simulink model "pendolo_simulink"  (R2026a)
settings: Solver=ode45  StopTime=30  MaxStep=0.01
values from neighbouring files (symbols this model uses):
  b = 0.2    [parametri_pendolo.m]
  ell = L/2    (= 0.5)    [parametri_pendolo.m]
  g = 9.81    [parametri_pendolo.m]
  I = m*L^2/3    (= 0.333333333333)    [parametri_pendolo.m]
  m = 1    [parametri_pendolo.m]
  omega0 = 0    [parametri_pendolo.m]
  theta0 = pi - 0.01    (= 3.13159265359)    [parametri_pendolo.m]
settings Model: Creator=bellu  LastModifiedBy=bellu

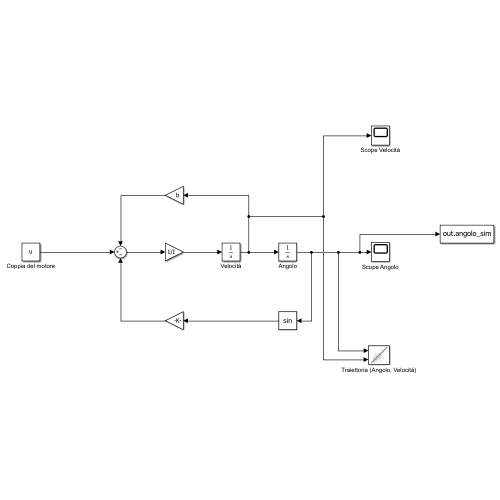
[thumbnail: Simulink's stored preview of the top-level diagram]
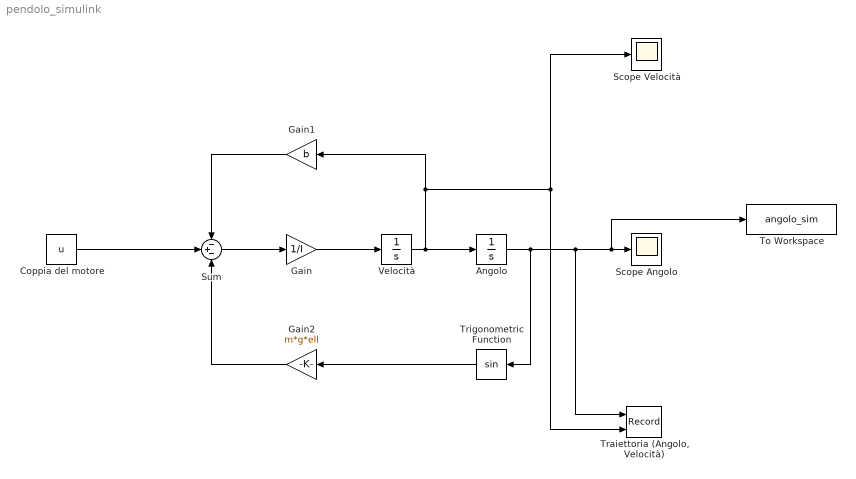
== system pendolo_simulink ==
  Angolo : Integrator  InitialCondition=theta0
  Coppia del motore : Constant  Value=u
  Gain : Gain  Gain=1/I
  Gain1 : Gain  Gain=b
  Gain2 : Gain  Gain=m*g*ell
  Scope Angolo : Scope
      settings: ActiveDisplayYMinimum=-3.4958404131067238  ActiveDisplayYMaximum=5.4026268178633838
  Scope Velocità : Scope
      settings: ActiveDisplayYMinimum=-7.8449946519179914  ActiveDisplayYMaximum=6.1158449546451417
  Sum : Sum  Inputs=-+-
  To Workspace : ToWorkspace  VariableName=angolo_sim  SaveFormat=Timeseries  SampleTime=-1
  "Traiettoria (Angolo, Velocità)" : Record  NumPorts=2.0  FileSettingsInternal="{\"entries\":[{\"content\":{\"excelSettings\":{\"content\":{},\"type\":\"Streamout.ExcelSettings\"},\"parquetSettings\":{\"content\":{},\"type\":\"Streamout.ParquetSettings\"}},\"type\":\"Streamout.FileSettingStorage\",\"uuid\":\"\"}],\"packageUris\":[\"http:\\/\\/schema.mathworks.com\\/mf0\\/streamout_blocks\\/R2020a\"],\"version\":\"1.0\"}"  FrameSettings=[0, 0]  Layout=[1 1]  SignalsInternal="{\"entries\":[{\"content\":{\"signals\":[{\"content\":{\"blockPath\":[],\"dimensions\":[1],\"domain\":\"\",\"lineColor\":\"#a2142f\",\"plots\":[ 1 ],\"port\":1,\"sid\":[\"\"],\"signalID\":1,\"signalName\":\"Angolo\"},\"type\":\"RecordBlkView.Signal\",\"uuid\":\"\"},{\"content\":{\"blockPath\":[],\"dimensions\":[1],\"domain\":\"\",\"lineColor\":\"#139fff\",\"plots\":[ 1 ],\"port\":2,\"sid\":[\"\"],\"signalID\":2,\"signalName\":\"Velocità\"},\"type\":\"RecordBlkView.Signal\",\"uuid\":\"\"}]},\"type\":\"RecordBlkView.InputSignals\",\"uuid\":\"\"}],\"packageUris\":[\"http:\\/\\/schema.mathworks.com\\/mf0\\/streamout_blocks\\/R2020a\"],\"version\":\"1.0\"}"  VisualizationBindings="{\"xyplotplugin\":{\"info\":[{\"series\":[{\"bindingParametersList\":[{\"parameter\":\"X-Axis\",\"signalID\":1,\"signalName\":\"Angolo\"},{\"parameter\":\"Y-Axis\",\"signalID\":2,\"signalName\":\"Velocità\"}],\"seriesID\":0},{\"bindingParametersList\":[{\"parameter\":\"X-Axis\",\"signalID\":1,\"signalName\":\"Angolo\"}],\"seriesID\":1}],\"subplotID\":1}]}}"  CompatibilityTag=XY
  Trigonometric Function : Trigonometry
  Velocità : Integrator  InitialCondition=omega0
  wires:
  Coppia del motore/1 -> Sum/2
  Sum/1 -> Gain/1
  Angolo/1 -> Trigonometric Function/1, "Traiettoria (Angolo, Velocità)"/1, To Workspace/1, Scope Angolo/1
  Gain/1 -> Velocità/1
  Gain1/1 -> Sum/1
  Trigonometric Function/1 -> Gain2/1
  Gain2/1 -> Sum/3
  Velocità/1 -> "Traiettoria (Angolo, Velocità)"/2, Scope Velocità/1, Gain1/1, Angolo/1
